simulink model "MTE484Lab3_a"  (R2024b)
settings: Solver=VariableStepAuto  StartTime=0.0  StopTime=200  RelTol=1e-3
settings Model: Creator=sebastianassuncao  LastModifiedBy=Alex V

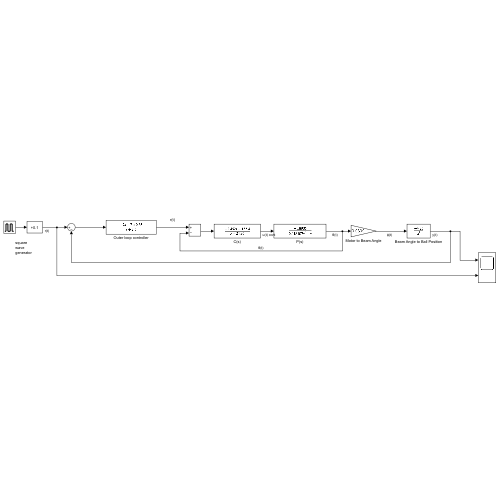
[thumbnail: Simulink's stored preview of the top-level diagram]
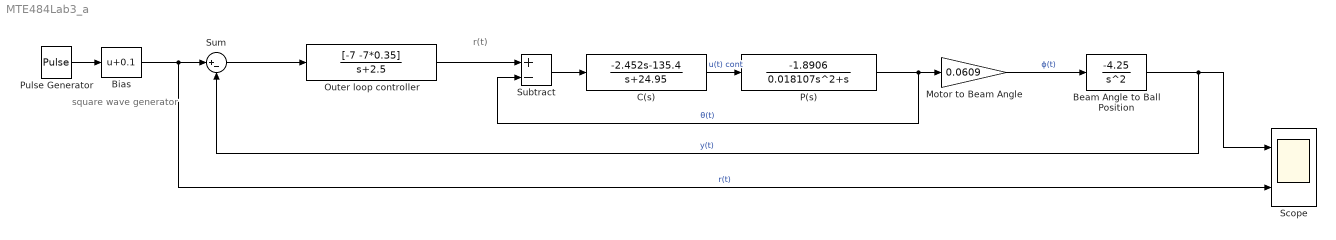
== system MTE484Lab3_a ==
  note: square
      | wave
      | generator
  note: r(t)
  Beam Angle to Ball Position : TransferFcn  Numerator=[-4.25]  Denominator=[1 0 0]
  Bias : Bias  Bias=0.1  SaturateOnIntegerOverflow=off
  C(s) : TransferFcn  Numerator=[-2.452 -135.4]  Denominator=[1 24.95]
  Motor to Beam Angle : Gain  Gain=0.0609
  Outer loop controller : TransferFcn  Numerator=[-7 -7*0.35]  Denominator=[1 2.5]
  P(s) : TransferFcn  Numerator=[-1.8906]  Denominator=[0.018107 1 0]
  Pulse Generator : DiscretePulseGenerator  PulseType=Time based  Amplitude=0.15  Period=50  PulseWidth=50
  Scope : Scope  NumInputPorts=2
  Subtract : Sum  Inputs=+-
  Sum : Sum  Inputs=|+-
  wires:
  P(s)/1 -> Motor to Beam Angle/1, Subtract/2  "θ(t)"
  Subtract/1 -> C(s)/1
  C(s)/1 -> P(s)/1  "u(t) cont"
  Pulse Generator/1 -> Bias/1
  Outer loop controller/1 -> Subtract/1
  Bias/1 -> Scope/2, Sum/1  "r(t)"
  Sum/1 -> Outer loop controller/1
  Motor to Beam Angle/1 -> Beam Angle to Ball Position/1  "ϕ(t)"
  Beam Angle to Ball Position/1 -> Scope/1, Sum/2  "y(t)"
